simulink model "sst_cllc_dcx"  (R2026b)
settings: Solver=ode23tb  StopTime=param.sim.simlength  FixedStep=tc  MaxStep=param.glb_time.tc
values from neighbouring files (symbols this model uses):
  param = struct()    [init_model.m]
undefined symbols (not defined in the file or in its folder): cllc_dcx_param_example
libraries: fl_lib x144, nesl_utility x71, mos_simple_2th_lib x8, discrete_time_low_pass_filter x2, lithium_ion_battery x1, cllc_dcx x1, single_phase_transformer x1, dab_single_phase_pwm_modulator x1, ee_lib x1
(part 3 of 4)

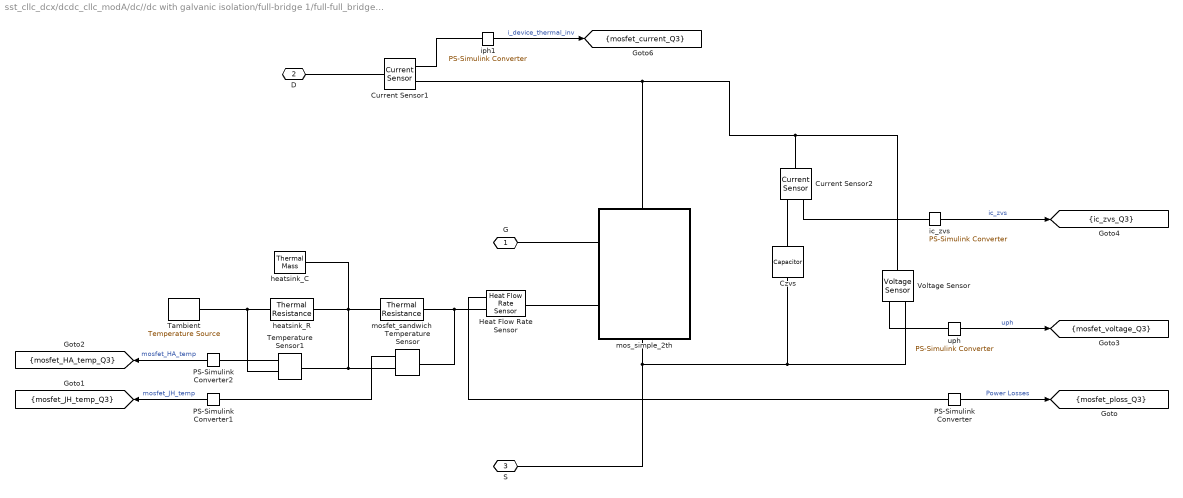
== system sst_cllc_dcx/dcdc_cllc_modA/dc//dc with galvanic isolation/full-bridge 1/full-full_bridge_ssc_mosfet_based/full_bridge_ssc_mosfet_based/mosfet_thermal_3 ==
  Current Sensor1 : fl_lib/Electrical/Electrical Sensors/Current Sensor
  Current Sensor2 : fl_lib/Electrical/Electrical Sensors/Current Sensor
  Czvs : fl_lib/Electrical/Electrical Elements/Capacitor  c=Csnubber_m F  r=Rsnubber_m Ohm  g=0 1/Ohm  i_specify=off  i_priority=None  i=0 A  i_nominal_specify=off  i_nominal_value=1  i_nominal_unit=A  v_specify=off  v_priority=None  v=0 V  v_nominal_specify=off  v_nominal_value=1  v_nominal_unit=V  vc_specify=off  vc_priority=High  vc=0 V  vc_nominal_specify=off  vc_nominal_value=1  vc_nominal_unit=V
  Heat Flow Rate Sensor : fl_lib/Thermal/Thermal Sensors/Heat Flow Rate Sensor
  PS-Simulink Converter : nesl_utility/PS-Simulink Converter  PhysicalDomain=network_engine_domain  SubClassName=ps_output  LeftPortType=input  RightPortType=output  PseudoPeriodic=off  Frequencies=[]  VectorFormat=1-D array  Unit=W  AffineConversion=off
  PS-Simulink Converter1 : nesl_utility/PS-Simulink Converter  PhysicalDomain=network_engine_domain  SubClassName=ps_output  LeftPortType=input  RightPortType=output  PseudoPeriodic=off  Frequencies=[]  VectorFormat=1-D array  Unit=degC  AffineConversion=off
  PS-Simulink Converter2 : nesl_utility/PS-Simulink Converter  PhysicalDomain=network_engine_domain  SubClassName=ps_output  LeftPortType=input  RightPortType=output  PseudoPeriodic=off  Frequencies=[]  VectorFormat=1-D array  Unit=degC  AffineConversion=off
  Tambient : fl_lib/Thermal/Thermal Sources/Temperature Source  temperature=Tambient_m degC
  Temperature Sensor : fl_lib/Thermal/Thermal Sensors/Temperature Sensor  temperature_measure=foundation.enum.MeasurementReference.difference
  Temperature Sensor1 : fl_lib/Thermal/Thermal Sensors/Temperature Sensor  temperature_measure=foundation.enum.MeasurementReference.difference
  Voltage Sensor : fl_lib/Electrical/Electrical Sensors/Voltage Sensor
  heatsink_C : fl_lib/Thermal/Thermal Elements/Thermal Mass  mass_type=foundation.enum.constant_variable.constant  mass=mass_heatsink_m kg  sp_heat=specific_heat_m J/(K*kg)  mass_min=1e-6 kg  num_ports=foundation.enum.numPorts2.one  m_specify=off  m_priority=High  m=1 kg  m_nominal_specify=off  m_nominal_value=1  m_nominal_unit=kg  T_specify=on  T_priority=High  T=DThs_init_m+Tambient_m degC  T_nominal_specify=off  T_nominal_value=1  T_nominal_unit=K  Q_specify=off  Q_priority=High  Q=0 W  Q_nominal_specify=off  Q_nominal_value=1  Q_nominal_unit=W
  heatsink_R : fl_lib/Thermal/Thermal Elements/Thermal Resistance  resistance=rth_mosfet_HA_m K/W  T_specify=off  T_priority=High  T=0 deltadegC  T_nominal_specify=off  T_nominal_value=1  T_nominal_unit=K  Q_specify=off  Q_priority=None  Q=0 W  Q_nominal_specify=off  Q_nominal_value=1  Q_nominal_unit=W
  ic_zvs : nesl_utility/PS-Simulink Converter  PhysicalDomain=network_engine_domain  SubClassName=ps_output  LeftPortType=input  RightPortType=output  PseudoPeriodic=off  Frequencies=[]  VectorFormat=1-D array  Unit=A  AffineConversion=off
  iph1 : nesl_utility/PS-Simulink Converter  PhysicalDomain=network_engine_domain  SubClassName=ps_output  LeftPortType=input  RightPortType=output  PseudoPeriodic=off  Frequencies=[]  VectorFormat=1-D array  Unit=A  AffineConversion=off
  mos_simple_2th : Subsystem
      settings: PortSchema="{\"entries\":[{\"content\":{\"sides\":[{\"content\":{\"connectorIds\":[\"LConn1\",\"LConn2\"]},\"type\":\"ConnectorPlacement.EquallySpacedRectSide\",\"uuid\":\"0c7df1d1-e739-4cca-908e-e4e85a8d5110\"},{\"content\":{\"side\":\"RIGHT\"},\"type\":\"ConnectorPlacement.EquallySpacedRectSide\",\"uuid\":\"6e0178b8-4891-4b94-aab6-d38b52a6c94b\"},{\"content\":{\"connectorIds\":[\"LConn3\"],\"side\":\"TOP\"},\"type\":\"ConnectorPlacement.EquallySpacedRectSide\",\"uuid\":\"66a82ce3-a212-45ef-89fa-79c9554ad3a2\"},{\"content\":{\"connectorIds\":[\"RConn1\"],\"side\":\"BOTTOM\"},\"type\":\"ConnectorPlacement.EquallySpacedRectSide\",\"uuid\":\"30e3dab1-9356-4de4-b881-b8bc9cf47aa5\"}]},\"type\":\"ConnectorPlacement.EquallySpacedConnector\",\"uuid\":\"69805b64-ad78-46b1-90c4-7e7bc5808829\"}],\"packageUris\":[\"http://schema.mathworks.com/mf0/Connector/R2020b\"],\"version\":\"1.0\"}"
  mosfet_sandwich : fl_lib/Thermal/Thermal Elements/Thermal Resistance  resistance=rth_mosfet_JH_m K/W  T_specify=off  T_priority=High  T=0 degC  T_nominal_specify=off  T_nominal_value=1  T_nominal_unit=K  Q_specify=off  Q_priority=None  Q=0 W  Q_nominal_specify=off  Q_nominal_value=1  Q_nominal_unit=W
  uph : nesl_utility/PS-Simulink Converter  PhysicalDomain=network_engine_domain  SubClassName=ps_output  LeftPortType=input  RightPortType=output  PseudoPeriodic=off  Frequencies=[]  VectorFormat=1-D array  Unit=V  AffineConversion=off
  G : PMIOPort  Side=Left
  D : PMIOPort  Port=2  Side=Left
  S : PMIOPort  Port=3  Side=Right
  tag scope: ic_zvs_Q3=scoped, mosfet_HA_temp_Q3=scoped, mosfet_JH_temp_Q3=scoped, mosfet_current_Q3=scoped, mosfet_ploss_Q3=scoped, mosfet_voltage_Q3=scoped
  wires:
  ic_zvs/1 -> [ic_zvs_Q3]  "ic_zvs"
  uph/1 -> [mosfet_voltage_Q3]  "uph"
  iph1/1 -> [mosfet_current_Q3]  "i_device_thermal_inv"
  PS-Simulink Converter1/1 -> [mosfet_JH_temp_Q3]  "mosfet_JH_temp"
  PS-Simulink Converter2/1 -> [mosfet_HA_temp_Q3]  "mosfet_HA_temp"
  PS-Simulink Converter/1 -> [mosfet_ploss_Q3]  "Power Losses"
  connections:
  Current Sensor2/RConn1 -- ic_zvs/LConn1
  Czvs/LConn1 -- Current Sensor2/RConn2
  Voltage Sensor/RConn1 -- uph/LConn1
  Current Sensor1/RConn1 -- iph1/LConn1
  Voltage Sensor/LConn1 -- Current Sensor1/RConn2 -- mos_simple_2th/LConn3 -- Current Sensor2/LConn1
  Current Sensor1/LConn1 -- D/RConn1
  mos_simple_2th/LConn2 -- Heat Flow Rate Sensor/LConn1
  Temperature Sensor1/RConn2 -- PS-Simulink Converter2/LConn1
  heatsink_R/RConn1 -- Tambient/LConn1 -- Temperature Sensor1/RConn1
  Temperature Sensor/RConn2 -- PS-Simulink Converter1/LConn1
  mosfet_sandwich/RConn1 -- heatsink_C/LConn1 -- heatsink_R/LConn1 -- Temperature Sensor/RConn1 -- Temperature Sensor1/LConn1
  Heat Flow Rate Sensor/RConn2 -- mosfet_sandwich/LConn1 -- Temperature Sensor/LConn1
  PS-Simulink Converter/LConn1 -- Heat Flow Rate Sensor/RConn1
  mos_simple_2th/LConn1 -- G/RConn1
  Voltage Sensor/RConn2 -- Czvs/RConn1 -- S/RConn1 -- mos_simple_2th/RConn1

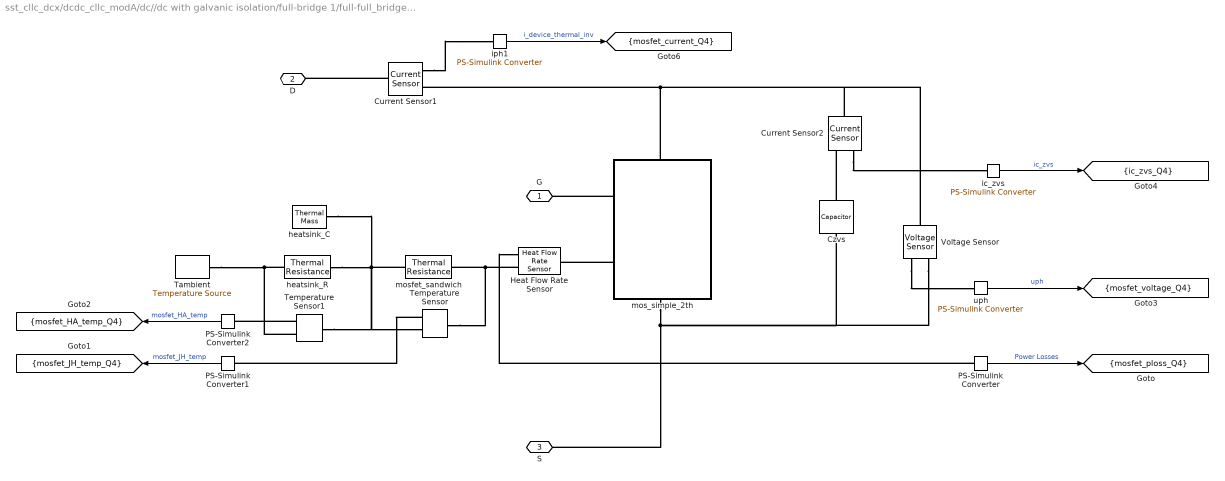
== system sst_cllc_dcx/dcdc_cllc_modA/dc//dc with galvanic isolation/full-bridge 1/full-full_bridge_ssc_mosfet_based/full_bridge_ssc_mosfet_based/mosfet_thermal_4 ==
  Current Sensor1 : fl_lib/Electrical/Electrical Sensors/Current Sensor
  Current Sensor2 : fl_lib/Electrical/Electrical Sensors/Current Sensor
  Czvs : fl_lib/Electrical/Electrical Elements/Capacitor  c=Csnubber_m F  r=Rsnubber_m Ohm  g=0 1/Ohm  i_specify=off  i_priority=None  i=0 A  i_nominal_specify=off  i_nominal_value=1  i_nominal_unit=A  v_specify=off  v_priority=None  v=0 V  v_nominal_specify=off  v_nominal_value=1  v_nominal_unit=V  vc_specify=off  vc_priority=High  vc=0 V  vc_nominal_specify=off  vc_nominal_value=1  vc_nominal_unit=V
  Heat Flow Rate Sensor : fl_lib/Thermal/Thermal Sensors/Heat Flow Rate Sensor
  PS-Simulink Converter : nesl_utility/PS-Simulink Converter  PhysicalDomain=network_engine_domain  SubClassName=ps_output  LeftPortType=input  RightPortType=output  PseudoPeriodic=off  Frequencies=[]  VectorFormat=1-D array  Unit=W  AffineConversion=off
  PS-Simulink Converter1 : nesl_utility/PS-Simulink Converter  PhysicalDomain=network_engine_domain  SubClassName=ps_output  LeftPortType=input  RightPortType=output  PseudoPeriodic=off  Frequencies=[]  VectorFormat=1-D array  Unit=degC  AffineConversion=off
  PS-Simulink Converter2 : nesl_utility/PS-Simulink Converter  PhysicalDomain=network_engine_domain  SubClassName=ps_output  LeftPortType=input  RightPortType=output  PseudoPeriodic=off  Frequencies=[]  VectorFormat=1-D array  Unit=degC  AffineConversion=off
  Tambient : fl_lib/Thermal/Thermal Sources/Temperature Source  temperature=Tambient_m degC
  Temperature Sensor : fl_lib/Thermal/Thermal Sensors/Temperature Sensor  temperature_measure=foundation.enum.MeasurementReference.difference
  Temperature Sensor1 : fl_lib/Thermal/Thermal Sensors/Temperature Sensor  temperature_measure=foundation.enum.MeasurementReference.difference
  Voltage Sensor : fl_lib/Electrical/Electrical Sensors/Voltage Sensor
  heatsink_C : fl_lib/Thermal/Thermal Elements/Thermal Mass  mass_type=foundation.enum.constant_variable.constant  mass=mass_heatsink_m kg  sp_heat=specific_heat_m J/(K*kg)  mass_min=1e-6 kg  num_ports=foundation.enum.numPorts2.one  m_specify=off  m_priority=High  m=1 kg  m_nominal_specify=off  m_nominal_value=1  m_nominal_unit=kg  T_specify=on  T_priority=High  T=DThs_init_m+Tambient_m degC  T_nominal_specify=off  T_nominal_value=1  T_nominal_unit=K  Q_specify=off  Q_priority=High  Q=0 W  Q_nominal_specify=off  Q_nominal_value=1  Q_nominal_unit=W
  heatsink_R : fl_lib/Thermal/Thermal Elements/Thermal Resistance  resistance=rth_mosfet_HA_m K/W  T_specify=off  T_priority=High  T=0 deltadegC  T_nominal_specify=off  T_nominal_value=1  T_nominal_unit=K  Q_specify=off  Q_priority=None  Q=0 W  Q_nominal_specify=off  Q_nominal_value=1  Q_nominal_unit=W
  ic_zvs : nesl_utility/PS-Simulink Converter  PhysicalDomain=network_engine_domain  SubClassName=ps_output  LeftPortType=input  RightPortType=output  PseudoPeriodic=off  Frequencies=[]  VectorFormat=1-D array  Unit=A  AffineConversion=off
  iph1 : nesl_utility/PS-Simulink Converter  PhysicalDomain=network_engine_domain  SubClassName=ps_output  LeftPortType=input  RightPortType=output  PseudoPeriodic=off  Frequencies=[]  VectorFormat=1-D array  Unit=A  AffineConversion=off
  mos_simple_2th : Subsystem
      settings: PortSchema="{\"entries\":[{\"content\":{\"sides\":[{\"content\":{\"connectorIds\":[\"LConn1\",\"LConn2\"]},\"type\":\"ConnectorPlacement.EquallySpacedRectSide\",\"uuid\":\"0c7df1d1-e739-4cca-908e-e4e85a8d5110\"},{\"content\":{\"side\":\"RIGHT\"},\"type\":\"ConnectorPlacement.EquallySpacedRectSide\",\"uuid\":\"6e0178b8-4891-4b94-aab6-d38b52a6c94b\"},{\"content\":{\"connectorIds\":[\"LConn3\"],\"side\":\"TOP\"},\"type\":\"ConnectorPlacement.EquallySpacedRectSide\",\"uuid\":\"66a82ce3-a212-45ef-89fa-79c9554ad3a2\"},{\"content\":{\"connectorIds\":[\"RConn1\"],\"side\":\"BOTTOM\"},\"type\":\"ConnectorPlacement.EquallySpacedRectSide\",\"uuid\":\"30e3dab1-9356-4de4-b881-b8bc9cf47aa5\"}]},\"type\":\"ConnectorPlacement.EquallySpacedConnector\",\"uuid\":\"69805b64-ad78-46b1-90c4-7e7bc5808829\"}],\"packageUris\":[\"http://schema.mathworks.com/mf0/Connector/R2020b\"],\"version\":\"1.0\"}"
  mosfet_sandwich : fl_lib/Thermal/Thermal Elements/Thermal Resistance  resistance=rth_mosfet_JH_m K/W  T_specify=off  T_priority=High  T=0 degC  T_nominal_specify=off  T_nominal_value=1  T_nominal_unit=K  Q_specify=off  Q_priority=None  Q=0 W  Q_nominal_specify=off  Q_nominal_value=1  Q_nominal_unit=W
  uph : nesl_utility/PS-Simulink Converter  PhysicalDomain=network_engine_domain  SubClassName=ps_output  LeftPortType=input  RightPortType=output  PseudoPeriodic=off  Frequencies=[]  VectorFormat=1-D array  Unit=V  AffineConversion=off
  G : PMIOPort  Side=Left
  D : PMIOPort  Port=2  Side=Left
  S : PMIOPort  Port=3  Side=Right
  tag scope: ic_zvs_Q4=scoped, mosfet_HA_temp_Q4=scoped, mosfet_JH_temp_Q4=scoped, mosfet_current_Q4=scoped, mosfet_ploss_Q4=scoped, mosfet_voltage_Q4=scoped
  wires:
  ic_zvs/1 -> [ic_zvs_Q4]  "ic_zvs"
  PS-Simulink Converter/1 -> [mosfet_ploss_Q4]  "Power Losses"
  PS-Simulink Converter2/1 -> [mosfet_HA_temp_Q4]  "mosfet_HA_temp"
  PS-Simulink Converter1/1 -> [mosfet_JH_temp_Q4]  "mosfet_JH_temp"
  iph1/1 -> [mosfet_current_Q4]  "i_device_thermal_inv"
  uph/1 -> [mosfet_voltage_Q4]  "uph"
  connections:
  Current Sensor2/RConn1 -- ic_zvs/LConn1
  Czvs/LConn1 -- Current Sensor2/RConn2
  Czvs/RConn1 -- Voltage Sensor/RConn2 -- mos_simple_2th/RConn1 -- S/RConn1
  mos_simple_2th/LConn1 -- G/RConn1
  PS-Simulink Converter/LConn1 -- Heat Flow Rate Sensor/RConn1
  Temperature Sensor/LConn1 -- mosfet_sandwich/LConn1 -- Heat Flow Rate Sensor/RConn2
  mosfet_sandwich/RConn1 -- heatsink_C/LConn1 -- heatsink_R/LConn1 -- Temperature Sensor1/LConn1 -- Temperature Sensor/RConn1
  Temperature Sensor/RConn2 -- PS-Simulink Converter1/LConn1
  heatsink_R/RConn1 -- Tambient/LConn1 -- Temperature Sensor1/RConn1
  Temperature Sensor1/RConn2 -- PS-Simulink Converter2/LConn1
  mos_simple_2th/LConn2 -- Heat Flow Rate Sensor/LConn1
  Current Sensor1/LConn1 -- D/RConn1
  Current Sensor2/LConn1 -- Voltage Sensor/LConn1 -- mos_simple_2th/LConn3 -- Current Sensor1/RConn2
  Current Sensor1/RConn1 -- iph1/LConn1
  Voltage Sensor/RConn1 -- uph/LConn1

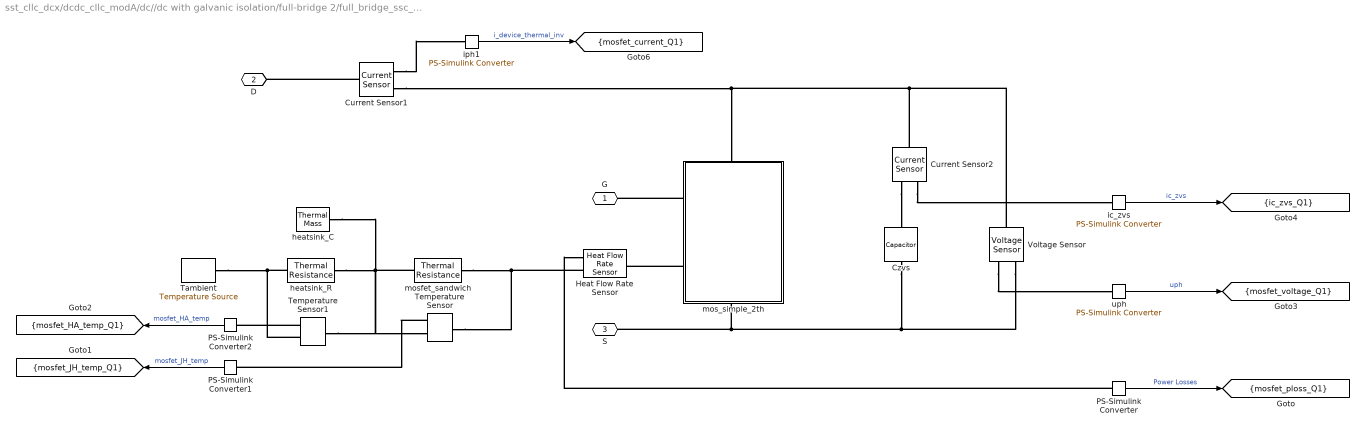
== system sst_cllc_dcx/dcdc_cllc_modA/dc//dc with galvanic isolation/full-bridge 2/full_bridge_ssc_mosfet_based/full_bridge_ssc_mosfet_based/mosfet_thermal_1 ==
  Current Sensor1 : fl_lib/Electrical/Electrical Sensors/Current Sensor
  Current Sensor2 : fl_lib/Electrical/Electrical Sensors/Current Sensor
  Czvs : fl_lib/Electrical/Electrical Elements/Capacitor  c=Csnubber_m F  r=Rsnubber_m Ohm  g=0 1/Ohm  i_specify=off  i_priority=None  i=0 A  i_nominal_specify=off  i_nominal_value=1  i_nominal_unit=A  v_specify=off  v_priority=None  v=0 V  v_nominal_specify=off  v_nominal_value=1  v_nominal_unit=V  vc_specify=off  vc_priority=High  vc=0 V  vc_nominal_specify=off  vc_nominal_value=1  vc_nominal_unit=V
  Heat Flow Rate Sensor : fl_lib/Thermal/Thermal Sensors/Heat Flow Rate Sensor
  PS-Simulink Converter : nesl_utility/PS-Simulink Converter  PhysicalDomain=network_engine_domain  SubClassName=ps_output  LeftPortType=input  RightPortType=output  PseudoPeriodic=off  Frequencies=[]  VectorFormat=1-D array  Unit=W  AffineConversion=off
  PS-Simulink Converter1 : nesl_utility/PS-Simulink Converter  PhysicalDomain=network_engine_domain  SubClassName=ps_output  LeftPortType=input  RightPortType=output  PseudoPeriodic=off  Frequencies=[]  VectorFormat=1-D array  Unit=degC  AffineConversion=off
  PS-Simulink Converter2 : nesl_utility/PS-Simulink Converter  PhysicalDomain=network_engine_domain  SubClassName=ps_output  LeftPortType=input  RightPortType=output  PseudoPeriodic=off  Frequencies=[]  VectorFormat=1-D array  Unit=degC  AffineConversion=off
  Tambient : fl_lib/Thermal/Thermal Sources/Temperature Source  temperature=Tambient_m degC
  Temperature Sensor : fl_lib/Thermal/Thermal Sensors/Temperature Sensor  temperature_measure=foundation.enum.MeasurementReference.difference
  Temperature Sensor1 : fl_lib/Thermal/Thermal Sensors/Temperature Sensor  temperature_measure=foundation.enum.MeasurementReference.difference
  Voltage Sensor : fl_lib/Electrical/Electrical Sensors/Voltage Sensor
  heatsink_C : fl_lib/Thermal/Thermal Elements/Thermal Mass  mass_type=foundation.enum.constant_variable.constant  mass=mass_heatsink_m kg  sp_heat=specific_heat_m J/(K*kg)  mass_min=1e-6 kg  num_ports=foundation.enum.numPorts2.one  m_specify=off  m_priority=High  m=1 kg  m_nominal_specify=off  m_nominal_value=1  m_nominal_unit=kg  T_specify=on  T_priority=High  T=DThs_init_m+Tambient_m degC  T_nominal_specify=off  T_nominal_value=1  T_nominal_unit=K  Q_specify=off  Q_priority=High  Q=0 W  Q_nominal_specify=off  Q_nominal_value=1  Q_nominal_unit=W
  heatsink_R : fl_lib/Thermal/Thermal Elements/Thermal Resistance  resistance=rth_mosfet_HA_m K/W  T_specify=off  T_priority=High  T=0 deltadegC  T_nominal_specify=off  T_nominal_value=1  T_nominal_unit=K  Q_specify=off  Q_priority=None  Q=0 W  Q_nominal_specify=off  Q_nominal_value=1  Q_nominal_unit=W
  ic_zvs : nesl_utility/PS-Simulink Converter  PhysicalDomain=network_engine_domain  SubClassName=ps_output  LeftPortType=input  RightPortType=output  PseudoPeriodic=off  Frequencies=[]  VectorFormat=1-D array  Unit=A  AffineConversion=off
  iph1 : nesl_utility/PS-Simulink Converter  PhysicalDomain=network_engine_domain  SubClassName=ps_output  LeftPortType=input  RightPortType=output  PseudoPeriodic=off  Frequencies=[]  VectorFormat=1-D array  Unit=A  AffineConversion=off
  mos_simple_2th : Subsystem
      settings: PortSchema="{\"entries\":[{\"content\":{\"sides\":[{\"content\":{\"connectorIds\":[\"LConn1\",\"LConn2\"]},\"type\":\"ConnectorPlacement.EquallySpacedRectSide\",\"uuid\":\"0c7df1d1-e739-4cca-908e-e4e85a8d5110\"},{\"content\":{\"side\":\"RIGHT\"},\"type\":\"ConnectorPlacement.EquallySpacedRectSide\",\"uuid\":\"6e0178b8-4891-4b94-aab6-d38b52a6c94b\"},{\"content\":{\"connectorIds\":[\"LConn3\"],\"side\":\"TOP\"},\"type\":\"ConnectorPlacement.EquallySpacedRectSide\",\"uuid\":\"66a82ce3-a212-45ef-89fa-79c9554ad3a2\"},{\"content\":{\"connectorIds\":[\"RConn1\"],\"side\":\"BOTTOM\"},\"type\":\"ConnectorPlacement.EquallySpacedRectSide\",\"uuid\":\"30e3dab1-9356-4de4-b881-b8bc9cf47aa5\"}]},\"type\":\"ConnectorPlacement.EquallySpacedConnector\",\"uuid\":\"69805b64-ad78-46b1-90c4-7e7bc5808829\"}],\"packageUris\":[\"http://schema.mathworks.com/mf0/Connector/R2020b\"],\"version\":\"1.0\"}"
  mosfet_sandwich : fl_lib/Thermal/Thermal Elements/Thermal Resistance  resistance=rth_mosfet_JH_m K/W  T_specify=off  T_priority=High  T=0 degC  T_nominal_specify=off  T_nominal_value=1  T_nominal_unit=K  Q_specify=off  Q_priority=None  Q=0 W  Q_nominal_specify=off  Q_nominal_value=1  Q_nominal_unit=W
  uph : nesl_utility/PS-Simulink Converter  PhysicalDomain=network_engine_domain  SubClassName=ps_output  LeftPortType=input  RightPortType=output  PseudoPeriodic=off  Frequencies=[]  VectorFormat=1-D array  Unit=V  AffineConversion=off
  G : PMIOPort  Side=Left
  D : PMIOPort  Port=2  Side=Left
  S : PMIOPort  Port=3  Side=Right
  tag scope: ic_zvs_Q1=scoped, mosfet_HA_temp_Q1=scoped, mosfet_JH_temp_Q1=scoped, mosfet_current_Q1=scoped, mosfet_ploss_Q1=scoped, mosfet_voltage_Q1=scoped
  wires:
  ic_zvs/1 -> [ic_zvs_Q1]  "ic_zvs"
  uph/1 -> [mosfet_voltage_Q1]  "uph"
  iph1/1 -> [mosfet_current_Q1]  "i_device_thermal_inv"
  PS-Simulink Converter1/1 -> [mosfet_JH_temp_Q1]  "mosfet_JH_temp"
  PS-Simulink Converter2/1 -> [mosfet_HA_temp_Q1]  "mosfet_HA_temp"
  PS-Simulink Converter/1 -> [mosfet_ploss_Q1]  "Power Losses"
  connections:
  Current Sensor2/RConn1 -- ic_zvs/LConn1
  Current Sensor2/RConn2 -- Czvs/LConn1
  Voltage Sensor/RConn1 -- uph/LConn1
  Current Sensor1/RConn1 -- iph1/LConn1
  Voltage Sensor/LConn1 -- Current Sensor2/LConn1 -- Current Sensor1/RConn2 -- mos_simple_2th/LConn3
  Current Sensor1/LConn1 -- D/RConn1
  mos_simple_2th/LConn2 -- Heat Flow Rate Sensor/LConn1
  Temperature Sensor1/RConn2 -- PS-Simulink Converter2/LConn1
  Temperature Sensor1/RConn1 -- heatsink_R/RConn1 -- Tambient/LConn1
  Temperature Sensor/RConn2 -- PS-Simulink Converter1/LConn1
  heatsink_C/LConn1 -- heatsink_R/LConn1 -- mosfet_sandwich/RConn1 -- Temperature Sensor/RConn1 -- Temperature Sensor1/LConn1
  Heat Flow Rate Sensor/RConn2 -- mosfet_sandwich/LConn1 -- Temperature Sensor/LConn1
  PS-Simulink Converter/LConn1 -- Heat Flow Rate Sensor/RConn1
  mos_simple_2th/LConn1 -- G/RConn1
  Voltage Sensor/RConn2 -- S/RConn1 -- mos_simple_2th/RConn1 -- Czvs/RConn1

== system sst_cllc_dcx/dcdc_cllc_modA/dc//dc with galvanic isolation/full-bridge 2/full_bridge_ssc_mosfet_based/full_bridge_ssc_mosfet_based/mosfet_thermal_2 ==
  Current Sensor1 : fl_lib/Electrical/Electrical Sensors/Current Sensor
  Current Sensor2 : fl_lib/Electrical/Electrical Sensors/Current Sensor
  Czvs : fl_lib/Electrical/Electrical Elements/Capacitor  c=Csnubber_m F  r=Rsnubber_m Ohm  g=0 1/Ohm  i_specify=off  i_priority=None  i=0 A  i_nominal_specify=off  i_nominal_value=1  i_nominal_unit=A  v_specify=off  v_priority=None  v=0 V  v_nominal_specify=off  v_nominal_value=1  v_nominal_unit=V  vc_specify=off  vc_priority=High  vc=0 V  vc_nominal_specify=off  vc_nominal_value=1  vc_nominal_unit=V
  Heat Flow Rate Sensor : fl_lib/Thermal/Thermal Sensors/Heat Flow Rate Sensor
  PS-Simulink Converter : nesl_utility/PS-Simulink Converter  PhysicalDomain=network_engine_domain  SubClassName=ps_output  LeftPortType=input  RightPortType=output  PseudoPeriodic=off  Frequencies=[]  VectorFormat=1-D array  Unit=W  AffineConversion=off
  PS-Simulink Converter1 : nesl_utility/PS-Simulink Converter  PhysicalDomain=network_engine_domain  SubClassName=ps_output  LeftPortType=input  RightPortType=output  PseudoPeriodic=off  Frequencies=[]  VectorFormat=1-D array  Unit=degC  AffineConversion=off
  PS-Simulink Converter2 : nesl_utility/PS-Simulink Converter  PhysicalDomain=network_engine_domain  SubClassName=ps_output  LeftPortType=input  RightPortType=output  PseudoPeriodic=off  Frequencies=[]  VectorFormat=1-D array  Unit=degC  AffineConversion=off
  Tambient : fl_lib/Thermal/Thermal Sources/Temperature Source  temperature=Tambient_m degC
  Temperature Sensor : fl_lib/Thermal/Thermal Sensors/Temperature Sensor  temperature_measure=foundation.enum.MeasurementReference.difference
  Temperature Sensor1 : fl_lib/Thermal/Thermal Sensors/Temperature Sensor  temperature_measure=foundation.enum.MeasurementReference.difference
  Voltage Sensor : fl_lib/Electrical/Electrical Sensors/Voltage Sensor
  heatsink_C : fl_lib/Thermal/Thermal Elements/Thermal Mass  mass_type=foundation.enum.constant_variable.constant  mass=mass_heatsink_m kg  sp_heat=specific_heat_m J/(K*kg)  mass_min=1e-6 kg  num_ports=foundation.enum.numPorts2.one  m_specify=off  m_priority=High  m=1 kg  m_nominal_specify=off  m_nominal_value=1  m_nominal_unit=kg  T_specify=on  T_priority=High  T=DThs_init_m+Tambient_m degC  T_nominal_specify=off  T_nominal_value=1  T_nominal_unit=K  Q_specify=off  Q_priority=High  Q=0 W  Q_nominal_specify=off  Q_nominal_value=1  Q_nominal_unit=W
  heatsink_R : fl_lib/Thermal/Thermal Elements/Thermal Resistance  resistance=rth_mosfet_HA_m K/W  T_specify=off  T_priority=High  T=0 deltadegC  T_nominal_specify=off  T_nominal_value=1  T_nominal_unit=K  Q_specify=off  Q_priority=None  Q=0 W  Q_nominal_specify=off  Q_nominal_value=1  Q_nominal_unit=W
  ic_zvs : nesl_utility/PS-Simulink Converter  PhysicalDomain=network_engine_domain  SubClassName=ps_output  LeftPortType=input  RightPortType=output  PseudoPeriodic=off  Frequencies=[]  VectorFormat=1-D array  Unit=A  AffineConversion=off
  iph1 : nesl_utility/PS-Simulink Converter  PhysicalDomain=network_engine_domain  SubClassName=ps_output  LeftPortType=input  RightPortType=output  PseudoPeriodic=off  Frequencies=[]  VectorFormat=1-D array  Unit=A  AffineConversion=off
  mos_simple_2th : Subsystem
      settings: PortSchema="{\"entries\":[{\"content\":{\"sides\":[{\"content\":{\"connectorIds\":[\"LConn1\",\"LConn2\"]},\"type\":\"ConnectorPlacement.EquallySpacedRectSide\",\"uuid\":\"0c7df1d1-e739-4cca-908e-e4e85a8d5110\"},{\"content\":{\"side\":\"RIGHT\"},\"type\":\"ConnectorPlacement.EquallySpacedRectSide\",\"uuid\":\"6e0178b8-4891-4b94-aab6-d38b52a6c94b\"},{\"content\":{\"connectorIds\":[\"LConn3\"],\"side\":\"TOP\"},\"type\":\"ConnectorPlacement.EquallySpacedRectSide\",\"uuid\":\"66a82ce3-a212-45ef-89fa-79c9554ad3a2\"},{\"content\":{\"connectorIds\":[\"RConn1\"],\"side\":\"BOTTOM\"},\"type\":\"ConnectorPlacement.EquallySpacedRectSide\",\"uuid\":\"30e3dab1-9356-4de4-b881-b8bc9cf47aa5\"}]},\"type\":\"ConnectorPlacement.EquallySpacedConnector\",\"uuid\":\"69805b64-ad78-46b1-90c4-7e7bc5808829\"}],\"packageUris\":[\"http://schema.mathworks.com/mf0/Connector/R2020b\"],\"version\":\"1.0\"}"
  mosfet_sandwich : fl_lib/Thermal/Thermal Elements/Thermal Resistance  resistance=rth_mosfet_JH_m K/W  T_specify=off  T_priority=High  T=0 degC  T_nominal_specify=off  T_nominal_value=1  T_nominal_unit=K  Q_specify=off  Q_priority=None  Q=0 W  Q_nominal_specify=off  Q_nominal_value=1  Q_nominal_unit=W
  uph : nesl_utility/PS-Simulink Converter  PhysicalDomain=network_engine_domain  SubClassName=ps_output  LeftPortType=input  RightPortType=output  PseudoPeriodic=off  Frequencies=[]  VectorFormat=1-D array  Unit=V  AffineConversion=off
  G : PMIOPort  Side=Left
  D : PMIOPort  Port=2  Side=Left
  S : PMIOPort  Port=3  Side=Right
  tag scope: ic_zvs_Q2=scoped, mosfet_HA_temp_Q2=scoped, mosfet_JH_temp_Q2=scoped, mosfet_current_Q2=scoped, mosfet_ploss_Q2=scoped, mosfet_voltage_Q2=scoped
  wires:
  ic_zvs/1 -> [ic_zvs_Q2]  "ic_zvs"
  PS-Simulink Converter/1 -> [mosfet_ploss_Q2]  "Power Losses"
  PS-Simulink Converter2/1 -> [mosfet_HA_temp_Q2]  "mosfet_HA_temp"
  PS-Simulink Converter1/1 -> [mosfet_JH_temp_Q2]  "mosfet_JH_temp"
  iph1/1 -> [mosfet_current_Q2]  "i_device_thermal_inv"
  uph/1 -> [mosfet_voltage_Q2]  "uph"
  connections:
  Current Sensor2/RConn1 -- ic_zvs/LConn1
  Czvs/LConn1 -- Current Sensor2/RConn2
  Czvs/RConn1 -- mos_simple_2th/RConn1 -- S/RConn1 -- Voltage Sensor/RConn2
  mos_simple_2th/LConn1 -- G/RConn1
  PS-Simulink Converter/LConn1 -- Heat Flow Rate Sensor/RConn1
  Temperature Sensor/LConn1 -- mosfet_sandwich/LConn1 -- Heat Flow Rate Sensor/RConn2
  heatsink_R/LConn1 -- heatsink_C/LConn1 -- mosfet_sandwich/RConn1 -- Temperature Sensor/RConn1 -- Temperature Sensor1/LConn1
  Temperature Sensor/RConn2 -- PS-Simulink Converter1/LConn1
  Tambient/LConn1 -- heatsink_R/RConn1 -- Temperature Sensor1/RConn1
  Temperature Sensor1/RConn2 -- PS-Simulink Converter2/LConn1
  mos_simple_2th/LConn2 -- Heat Flow Rate Sensor/LConn1
  Current Sensor1/LConn1 -- D/RConn1
  Current Sensor2/LConn1 -- Voltage Sensor/LConn1 -- mos_simple_2th/LConn3 -- Current Sensor1/RConn2
  Current Sensor1/RConn1 -- iph1/LConn1
  Voltage Sensor/RConn1 -- uph/LConn1

== system sst_cllc_dcx/dcdc_cllc_modA/dc//dc with galvanic isolation/full-bridge 2/full_bridge_ssc_mosfet_based/full_bridge_ssc_mosfet_based/mosfet_thermal_3 ==
  Current Sensor1 : fl_lib/Electrical/Electrical Sensors/Current Sensor
  Current Sensor2 : fl_lib/Electrical/Electrical Sensors/Current Sensor
  Czvs : fl_lib/Electrical/Electrical Elements/Capacitor  c=Csnubber_m F  r=Rsnubber_m Ohm  g=0 1/Ohm  i_specify=off  i_priority=None  i=0 A  i_nominal_specify=off  i_nominal_value=1  i_nominal_unit=A  v_specify=off  v_priority=None  v=0 V  v_nominal_specify=off  v_nominal_value=1  v_nominal_unit=V  vc_specify=off  vc_priority=High  vc=0 V  vc_nominal_specify=off  vc_nominal_value=1  vc_nominal_unit=V
  Heat Flow Rate Sensor : fl_lib/Thermal/Thermal Sensors/Heat Flow Rate Sensor
  PS-Simulink Converter : nesl_utility/PS-Simulink Converter  PhysicalDomain=network_engine_domain  SubClassName=ps_output  LeftPortType=input  RightPortType=output  PseudoPeriodic=off  Frequencies=[]  VectorFormat=1-D array  Unit=W  AffineConversion=off
  PS-Simulink Converter1 : nesl_utility/PS-Simulink Converter  PhysicalDomain=network_engine_domain  SubClassName=ps_output  LeftPortType=input  RightPortType=output  PseudoPeriodic=off  Frequencies=[]  VectorFormat=1-D array  Unit=degC  AffineConversion=off
  PS-Simulink Converter2 : nesl_utility/PS-Simulink Converter  PhysicalDomain=network_engine_domain  SubClassName=ps_output  LeftPortType=input  RightPortType=output  PseudoPeriodic=off  Frequencies=[]  VectorFormat=1-D array  Unit=degC  AffineConversion=off
  Tambient : fl_lib/Thermal/Thermal Sources/Temperature Source  temperature=Tambient_m degC
  Temperature Sensor : fl_lib/Thermal/Thermal Sensors/Temperature Sensor  temperature_measure=foundation.enum.MeasurementReference.difference
  Temperature Sensor1 : fl_lib/Thermal/Thermal Sensors/Temperature Sensor  temperature_measure=foundation.enum.MeasurementReference.difference
  Voltage Sensor : fl_lib/Electrical/Electrical Sensors/Voltage Sensor
  heatsink_C : fl_lib/Thermal/Thermal Elements/Thermal Mass  mass_type=foundation.enum.constant_variable.constant  mass=mass_heatsink_m kg  sp_heat=specific_heat_m J/(K*kg)  mass_min=1e-6 kg  num_ports=foundation.enum.numPorts2.one  m_specify=off  m_priority=High  m=1 kg  m_nominal_specify=off  m_nominal_value=1  m_nominal_unit=kg  T_specify=on  T_priority=High  T=DThs_init_m+Tambient_m degC  T_nominal_specify=off  T_nominal_value=1  T_nominal_unit=K  Q_specify=off  Q_priority=High  Q=0 W  Q_nominal_specify=off  Q_nominal_value=1  Q_nominal_unit=W
  heatsink_R : fl_lib/Thermal/Thermal Elements/Thermal Resistance  resistance=rth_mosfet_HA_m K/W  T_specify=off  T_priority=High  T=0 deltadegC  T_nominal_specify=off  T_nominal_value=1  T_nominal_unit=K  Q_specify=off  Q_priority=None  Q=0 W  Q_nominal_specify=off  Q_nominal_value=1  Q_nominal_unit=W
  ic_zvs : nesl_utility/PS-Simulink Converter  PhysicalDomain=network_engine_domain  SubClassName=ps_output  LeftPortType=input  RightPortType=output  PseudoPeriodic=off  Frequencies=[]  VectorFormat=1-D array  Unit=A  AffineConversion=off
  iph1 : nesl_utility/PS-Simulink Converter  PhysicalDomain=network_engine_domain  SubClassName=ps_output  LeftPortType=input  RightPortType=output  PseudoPeriodic=off  Frequencies=[]  VectorFormat=1-D array  Unit=A  AffineConversion=off
  mos_simple_2th : Subsystem
      settings: PortSchema="{\"entries\":[{\"content\":{\"sides\":[{\"content\":{\"connectorIds\":[\"LConn1\",\"LConn2\"]},\"type\":\"ConnectorPlacement.EquallySpacedRectSide\",\"uuid\":\"0c7df1d1-e739-4cca-908e-e4e85a8d5110\"},{\"content\":{\"side\":\"RIGHT\"},\"type\":\"ConnectorPlacement.EquallySpacedRectSide\",\"uuid\":\"6e0178b8-4891-4b94-aab6-d38b52a6c94b\"},{\"content\":{\"connectorIds\":[\"LConn3\"],\"side\":\"TOP\"},\"type\":\"ConnectorPlacement.EquallySpacedRectSide\",\"uuid\":\"66a82ce3-a212-45ef-89fa-79c9554ad3a2\"},{\"content\":{\"connectorIds\":[\"RConn1\"],\"side\":\"BOTTOM\"},\"type\":\"ConnectorPlacement.EquallySpacedRectSide\",\"uuid\":\"30e3dab1-9356-4de4-b881-b8bc9cf47aa5\"}]},\"type\":\"ConnectorPlacement.EquallySpacedConnector\",\"uuid\":\"69805b64-ad78-46b1-90c4-7e7bc5808829\"}],\"packageUris\":[\"http://schema.mathworks.com/mf0/Connector/R2020b\"],\"version\":\"1.0\"}"
  mosfet_sandwich : fl_lib/Thermal/Thermal Elements/Thermal Resistance  resistance=rth_mosfet_JH_m K/W  T_specify=off  T_priority=High  T=0 degC  T_nominal_specify=off  T_nominal_value=1  T_nominal_unit=K  Q_specify=off  Q_priority=None  Q=0 W  Q_nominal_specify=off  Q_nominal_value=1  Q_nominal_unit=W
  uph : nesl_utility/PS-Simulink Converter  PhysicalDomain=network_engine_domain  SubClassName=ps_output  LeftPortType=input  RightPortType=output  PseudoPeriodic=off  Frequencies=[]  VectorFormat=1-D array  Unit=V  AffineConversion=off
  G : PMIOPort  Side=Left
  D : PMIOPort  Port=2  Side=Left
  S : PMIOPort  Port=3  Side=Right
  tag scope: ic_zvs_Q3=scoped, mosfet_HA_temp_Q3=scoped, mosfet_JH_temp_Q3=scoped, mosfet_current_Q3=scoped, mosfet_ploss_Q3=scoped, mosfet_voltage_Q3=scoped
  wires:
  ic_zvs/1 -> [ic_zvs_Q3]  "ic_zvs"
  uph/1 -> [mosfet_voltage_Q3]  "uph"
  iph1/1 -> [mosfet_current_Q3]  "i_device_thermal_inv"
  PS-Simulink Converter1/1 -> [mosfet_JH_temp_Q3]  "mosfet_JH_temp"
  PS-Simulink Converter2/1 -> [mosfet_HA_temp_Q3]  "mosfet_HA_temp"
  PS-Simulink Converter/1 -> [mosfet_ploss_Q3]  "Power Losses"
  connections:
  Current Sensor2/RConn1 -- ic_zvs/LConn1
  Czvs/LConn1 -- Current Sensor2/RConn2
  Voltage Sensor/RConn1 -- uph/LConn1
  Current Sensor1/RConn1 -- iph1/LConn1
  Voltage Sensor/LConn1 -- mos_simple_2th/LConn3 -- Current Sensor1/RConn2 -- Current Sensor2/LConn1
  Current Sensor1/LConn1 -- D/RConn1
  mos_simple_2th/LConn2 -- Heat Flow Rate Sensor/LConn1
  Temperature Sensor1/RConn2 -- PS-Simulink Converter2/LConn1
  heatsink_R/RConn1 -- Tambient/LConn1 -- Temperature Sensor1/RConn1
  Temperature Sensor/RConn2 -- PS-Simulink Converter1/LConn1
  mosfet_sandwich/RConn1 -- heatsink_C/LConn1 -- heatsink_R/LConn1 -- Temperature Sensor/RConn1 -- Temperature Sensor1/LConn1
  Heat Flow Rate Sensor/RConn2 -- mosfet_sandwich/LConn1 -- Temperature Sensor/LConn1
  PS-Simulink Converter/LConn1 -- Heat Flow Rate Sensor/RConn1
  mos_simple_2th/LConn1 -- G/RConn1
  Voltage Sensor/RConn2 -- Czvs/RConn1 -- mos_simple_2th/RConn1 -- S/RConn1

== system sst_cllc_dcx/dcdc_cllc_modA/dc//dc with galvanic isolation/full-bridge 2/full_bridge_ssc_mosfet_based/full_bridge_ssc_mosfet_based/mosfet_thermal_4 ==
  Current Sensor1 : fl_lib/Electrical/Electrical Sensors/Current Sensor
  Current Sensor2 : fl_lib/Electrical/Electrical Sensors/Current Sensor
  Czvs : fl_lib/Electrical/Electrical Elements/Capacitor  c=Csnubber_m F  r=Rsnubber_m Ohm  g=0 1/Ohm  i_specify=off  i_priority=None  i=0 A  i_nominal_specify=off  i_nominal_value=1  i_nominal_unit=A  v_specify=off  v_priority=None  v=0 V  v_nominal_specify=off  v_nominal_value=1  v_nominal_unit=V  vc_specify=off  vc_priority=High  vc=0 V  vc_nominal_specify=off  vc_nominal_value=1  vc_nominal_unit=V
  Heat Flow Rate Sensor : fl_lib/Thermal/Thermal Sensors/Heat Flow Rate Sensor
  PS-Simulink Converter : nesl_utility/PS-Simulink Converter  PhysicalDomain=network_engine_domain  SubClassName=ps_output  LeftPortType=input  RightPortType=output  PseudoPeriodic=off  Frequencies=[]  VectorFormat=1-D array  Unit=W  AffineConversion=off
  PS-Simulink Converter1 : nesl_utility/PS-Simulink Converter  PhysicalDomain=network_engine_domain  SubClassName=ps_output  LeftPortType=input  RightPortType=output  PseudoPeriodic=off  Frequencies=[]  VectorFormat=1-D array  Unit=degC  AffineConversion=off
  PS-Simulink Converter2 : nesl_utility/PS-Simulink Converter  PhysicalDomain=network_engine_domain  SubClassName=ps_output  LeftPortType=input  RightPortType=output  PseudoPeriodic=off  Frequencies=[]  VectorFormat=1-D array  Unit=degC  AffineConversion=off
  Tambient : fl_lib/Thermal/Thermal Sources/Temperature Source  temperature=Tambient_m degC
  Temperature Sensor : fl_lib/Thermal/Thermal Sensors/Temperature Sensor  temperature_measure=foundation.enum.MeasurementReference.difference
  Temperature Sensor1 : fl_lib/Thermal/Thermal Sensors/Temperature Sensor  temperature_measure=foundation.enum.MeasurementReference.difference
  Voltage Sensor : fl_lib/Electrical/Electrical Sensors/Voltage Sensor
  heatsink_C : fl_lib/Thermal/Thermal Elements/Thermal Mass  mass_type=foundation.enum.constant_variable.constant  mass=mass_heatsink_m kg  sp_heat=specific_heat_m J/(K*kg)  mass_min=1e-6 kg  num_ports=foundation.enum.numPorts2.one  m_specify=off  m_priority=High  m=1 kg  m_nominal_specify=off  m_nominal_value=1  m_nominal_unit=kg  T_specify=on  T_priority=High  T=DThs_init_m+Tambient_m degC  T_nominal_specify=off  T_nominal_value=1  T_nominal_unit=K  Q_specify=off  Q_priority=High  Q=0 W  Q_nominal_specify=off  Q_nominal_value=1  Q_nominal_unit=W
  heatsink_R : fl_lib/Thermal/Thermal Elements/Thermal Resistance  resistance=rth_mosfet_HA_m K/W  T_specify=off  T_priority=High  T=0 deltadegC  T_nominal_specify=off  T_nominal_value=1  T_nominal_unit=K  Q_specify=off  Q_priority=None  Q=0 W  Q_nominal_specify=off  Q_nominal_value=1  Q_nominal_unit=W
  ic_zvs : nesl_utility/PS-Simulink Converter  PhysicalDomain=network_engine_domain  SubClassName=ps_output  LeftPortType=input  RightPortType=output  PseudoPeriodic=off  Frequencies=[]  VectorFormat=1-D array  Unit=A  AffineConversion=off
  iph1 : nesl_utility/PS-Simulink Converter  PhysicalDomain=network_engine_domain  SubClassName=ps_output  LeftPortType=input  RightPortType=output  PseudoPeriodic=off  Frequencies=[]  VectorFormat=1-D array  Unit=A  AffineConversion=off
  mos_simple_2th : Subsystem
      settings: PortSchema="{\"entries\":[{\"content\":{\"sides\":[{\"content\":{\"connectorIds\":[\"LConn1\",\"LConn2\"]},\"type\":\"ConnectorPlacement.EquallySpacedRectSide\",\"uuid\":\"0c7df1d1-e739-4cca-908e-e4e85a8d5110\"},{\"content\":{\"side\":\"RIGHT\"},\"type\":\"ConnectorPlacement.EquallySpacedRectSide\",\"uuid\":\"6e0178b8-4891-4b94-aab6-d38b52a6c94b\"},{\"content\":{\"connectorIds\":[\"LConn3\"],\"side\":\"TOP\"},\"type\":\"ConnectorPlacement.EquallySpacedRectSide\",\"uuid\":\"66a82ce3-a212-45ef-89fa-79c9554ad3a2\"},{\"content\":{\"connectorIds\":[\"RConn1\"],\"side\":\"BOTTOM\"},\"type\":\"ConnectorPlacement.EquallySpacedRectSide\",\"uuid\":\"30e3dab1-9356-4de4-b881-b8bc9cf47aa5\"}]},\"type\":\"ConnectorPlacement.EquallySpacedConnector\",\"uuid\":\"69805b64-ad78-46b1-90c4-7e7bc5808829\"}],\"packageUris\":[\"http://schema.mathworks.com/mf0/Connector/R2020b\"],\"version\":\"1.0\"}"
  mosfet_sandwich : fl_lib/Thermal/Thermal Elements/Thermal Resistance  resistance=rth_mosfet_JH_m K/W  T_specify=off  T_priority=High  T=0 degC  T_nominal_specify=off  T_nominal_value=1  T_nominal_unit=K  Q_specify=off  Q_priority=None  Q=0 W  Q_nominal_specify=off  Q_nominal_value=1  Q_nominal_unit=W
  uph : nesl_utility/PS-Simulink Converter  PhysicalDomain=network_engine_domain  SubClassName=ps_output  LeftPortType=input  RightPortType=output  PseudoPeriodic=off  Frequencies=[]  VectorFormat=1-D array  Unit=V  AffineConversion=off
  G : PMIOPort  Side=Left
  D : PMIOPort  Port=2  Side=Left
  S : PMIOPort  Port=3  Side=Right
  tag scope: ic_zvs_Q4=scoped, mosfet_HA_temp_Q4=scoped, mosfet_JH_temp_Q4=scoped, mosfet_current_Q4=scoped, mosfet_ploss_Q4=scoped, mosfet_voltage_Q4=scoped
  wires:
  ic_zvs/1 -> [ic_zvs_Q4]  "ic_zvs"
  PS-Simulink Converter/1 -> [mosfet_ploss_Q4]  "Power Losses"
  PS-Simulink Converter2/1 -> [mosfet_HA_temp_Q4]  "mosfet_HA_temp"
  PS-Simulink Converter1/1 -> [mosfet_JH_temp_Q4]  "mosfet_JH_temp"
  iph1/1 -> [mosfet_current_Q4]  "i_device_thermal_inv"
  uph/1 -> [mosfet_voltage_Q4]  "uph"
  connections:
  Current Sensor2/RConn1 -- ic_zvs/LConn1
  Czvs/LConn1 -- Current Sensor2/RConn2
  Czvs/RConn1 -- Voltage Sensor/RConn2 -- mos_simple_2th/RConn1 -- S/RConn1
  mos_simple_2th/LConn1 -- G/RConn1
  PS-Simulink Converter/LConn1 -- Heat Flow Rate Sensor/RConn1
  Temperature Sensor/LConn1 -- mosfet_sandwich/LConn1 -- Heat Flow Rate Sensor/RConn2
  mosfet_sandwich/RConn1 -- heatsink_C/LConn1 -- heatsink_R/LConn1 -- Temperature Sensor1/LConn1 -- Temperature Sensor/RConn1
  Temperature Sensor/RConn2 -- PS-Simulink Converter1/LConn1
  heatsink_R/RConn1 -- Tambient/LConn1 -- Temperature Sensor1/RConn1
  Temperature Sensor1/RConn2 -- PS-Simulink Converter2/LConn1
  mos_simple_2th/LConn2 -- Heat Flow Rate Sensor/LConn1
  Current Sensor1/LConn1 -- D/RConn1
  Current Sensor2/LConn1 -- Voltage Sensor/LConn1 -- mos_simple_2th/LConn3 -- Current Sensor1/RConn2
  Current Sensor1/RConn1 -- iph1/LConn1
  Voltage Sensor/RConn1 -- uph/LConn1

== system sst_cllc_dcx/dcdc_cllc_modA/dc//dc with galvanic isolation/full-bridge 1/full-full_bridge_ssc_mosfet_based/full_bridge_ssc_mosfet_based/mosfet_thermal_1/mos_simple_2th ==
  PS Terminator{,1..3} (4 alike) : fl_lib/Physical Signals/Sinks/PS Terminator
  mos_simple_2th : mos_simple_2th_lib/MOS_SIMPLE_2TH Simplified power MOSFET + antiparallel diode, two thermal ports  Rds_on=Rds_on_m Ohm  alpha_R=0 1/K  Tj_ref=398.15 K  Roff=1e7 Ohm  Vf=Vdon_diode_m V  Rd=Rdon_diode_m Ohm  two_die=1  G_th=0.5  Eon_ref=Eon_m J  Eoff_ref=Eoff_m J  Err_ref=0.5e-3 J  Iref=Ion_sw_loss_m A  Vref=Voff_sw_loss_m V  ki=1  kv=1  Vth_off=50 V  Vth_on=25 V  V_sm=10 V  tau_s=100e-9 s  tau_v=10e-6 s  tau_p=50e-6 s  i_eps=1e-3 A  v_eps=1e-3 V  v_specify=off  v_priority=None  v=0 V  v_nominal_specify=off  v_nominal_value=1  v_nominal_unit=V  i_specify=off  i_priority=None  i=0 A  i_nominal_specify=off  i_nominal_value=1  i_nominal_unit=A  ich_specify=off  ich_priority=None  ich=0 A  ich_nominal_specify=off  ich_nominal_value=1  ich_nominal_unit=A  ichp_specify=off  ichp_priority=None  ichp=0 A  ichp_nominal_specify=off  ichp_nominal_value=1  ichp_nominal_unit=A  idio_specify=off  idio_priority=None  idio=0 A  idio_nominal_specify=off  idio_nominal_value=1  idio_nominal_unit=A  vfd_specify=off  vfd_priority=None  vfd=0 V  vfd_nominal_specify=off  vfd_nominal_value=1  vfd_nominal_unit=V  ith_specify=off  ith_priority=None  ith=0 A  ith_nominal_specify=off  ith_nominal_value=1  ith_nominal_unit=A  idh_specify=off  idh_priority=None  idh=0 A  idh_nominal_specify=off  idh_nominal_value=1  idh_nominal_unit=A  vbl_specify=off  vbl_priority=None  vbl=600 V  vbl_nominal_specify=off  vbl_nominal_value=1  vbl_nominal_unit=V  hb_specify=off  hb_priority=None  hb=0  hb_nominal_specify=off  hb_nominal_value=1  hb_nominal_unit=1  Gch_specify=off  Gch_priority=None  Gch=0 S  Gch_nominal_specify=off  Gch_nominal_value=1  Gch_nominal_unit=S  gl_specify=off  gl_priority=None  gl=0  gl_nominal_specify=off  gl_nominal_value=1  gl_nominal_unit=1  Rds_specify=off  Rds_priority=None  Rds=1e-3 Ohm  Rds_nominal_specify=off  Rds_nominal_value=1  Rds_nominal_unit=Ohm  xr_specify=off  xr_priority=None  xr=1  xr_nominal_specify=off  xr_nominal_value=1  xr_nominal_unit=1  Eot_specify=off  Eot_priority=None  Eot=0 J  Eot_nominal_specify=off  Eot_nominal_value=1  Eot_nominal_unit=J  Eod_specify=off  Eod_priority=None  Eod=0 J  Eod_nominal_specify=off  Eod_nominal_value=1  Eod_nominal_unit=J  Pswt_specify=off  Pswt_priority=None  Pswt=0 W  Pswt_nominal_specify=off  Pswt_nominal_value=1  Pswt_nominal_unit=W  Pswd_specify=off  Pswd_priority=None  Pswd=0 W  Pswd_nominal_specify=off  Pswd_nominal_value=1  Pswd_nominal_unit=W  Pct_specify=off  Pct_priority=None  Pct=0 W  Pct_nominal_specify=off  Pct_nominal_value=1  Pct_nominal_unit=W  Pcd_specify=off  Pcd_priority=None  Pcd=0 W  Pcd_nominal_specify=off  Pcd_nominal_value=1  Pcd_nominal_unit=W  Qt_specify=off  Qt_priority=None  Qt=0 W  Qt_nominal_specify=off  Qt_nominal_value=1  Qt_nominal_unit=W  Qd_specify=off  Qd_priority=None  Qd=0 W  Qd_nominal_specify=off  Qd_nominal_value=1  Qd_nominal_unit=W  Eqt_specify=off  Eqt_priority=None  Eqt=0 J  Eqd_specify=off  Eqd_priority=None  Eqd=0 J
  G : PMIOPort  Side=Left
  H : PMIOPort  Port=2  Side=Left
  D : PMIOPort  Port=3  Side=Left
  S : PMIOPort  Port=4  Side=Right
  connections:
  mos_simple_2th/LConn1 -- D/RConn1
  mos_simple_2th/RConn1 -- S/RConn1
  mos_simple_2th/LConn3 -- G/RConn1
  mos_simple_2th/LConn2 -- mos_simple_2th/RConn2 -- H/RConn1
  PS Terminator/LConn1 -- mos_simple_2th/RConn3
  PS Terminator1/LConn1 -- mos_simple_2th/RConn4
  PS Terminator2/LConn1 -- mos_simple_2th/RConn5
  PS Terminator3/LConn1 -- mos_simple_2th/RConn6

== system sst_cllc_dcx/dcdc_cllc_modA/dc//dc with galvanic isolation/full-bridge 1/full-full_bridge_ssc_mosfet_based/full_bridge_ssc_mosfet_based/mosfet_thermal_2/mos_simple_2th ==
  PS Terminator{,1..3} (4 alike) : fl_lib/Physical Signals/Sinks/PS Terminator
  mos_simple_2th : mos_simple_2th_lib/MOS_SIMPLE_2TH Simplified power MOSFET + antiparallel diode, two thermal ports  Rds_on=Rds_on_m Ohm  alpha_R=0 1/K  Tj_ref=398.15 K  Roff=1e7 Ohm  Vf=Vdon_diode_m V  Rd=Rdon_diode_m Ohm  two_die=1  G_th=0.5  Eon_ref=Eon_m J  Eoff_ref=Eoff_m J  Err_ref=0.5e-3 J  Iref=Ion_sw_loss_m A  Vref=Voff_sw_loss_m V  ki=1  kv=1  Vth_off=50 V  Vth_on=25 V  V_sm=10 V  tau_s=100e-9 s  tau_v=10e-6 s  tau_p=50e-6 s  i_eps=1e-3 A  v_eps=1e-3 V  v_specify=off  v_priority=None  v=0 V  v_nominal_specify=off  v_nominal_value=1  v_nominal_unit=V  i_specify=off  i_priority=None  i=0 A  i_nominal_specify=off  i_nominal_value=1  i_nominal_unit=A  ich_specify=off  ich_priority=None  ich=0 A  ich_nominal_specify=off  ich_nominal_value=1  ich_nominal_unit=A  ichp_specify=off  ichp_priority=None  ichp=0 A  ichp_nominal_specify=off  ichp_nominal_value=1  ichp_nominal_unit=A  idio_specify=off  idio_priority=None  idio=0 A  idio_nominal_specify=off  idio_nominal_value=1  idio_nominal_unit=A  vfd_specify=off  vfd_priority=None  vfd=0 V  vfd_nominal_specify=off  vfd_nominal_value=1  vfd_nominal_unit=V  ith_specify=off  ith_priority=None  ith=0 A  ith_nominal_specify=off  ith_nominal_value=1  ith_nominal_unit=A  idh_specify=off  idh_priority=None  idh=0 A  idh_nominal_specify=off  idh_nominal_value=1  idh_nominal_unit=A  vbl_specify=off  vbl_priority=None  vbl=600 V  vbl_nominal_specify=off  vbl_nominal_value=1  vbl_nominal_unit=V  hb_specify=off  hb_priority=None  hb=0  hb_nominal_specify=off  hb_nominal_value=1  hb_nominal_unit=1  Gch_specify=off  Gch_priority=None  Gch=0 S  Gch_nominal_specify=off  Gch_nominal_value=1  Gch_nominal_unit=S  gl_specify=off  gl_priority=None  gl=0  gl_nominal_specify=off  gl_nominal_value=1  gl_nominal_unit=1  Rds_specify=off  Rds_priority=None  Rds=1e-3 Ohm  Rds_nominal_specify=off  Rds_nominal_value=1  Rds_nominal_unit=Ohm  xr_specify=off  xr_priority=None  xr=1  xr_nominal_specify=off  xr_nominal_value=1  xr_nominal_unit=1  Eot_specify=off  Eot_priority=None  Eot=0 J  Eot_nominal_specify=off  Eot_nominal_value=1  Eot_nominal_unit=J  Eod_specify=off  Eod_priority=None  Eod=0 J  Eod_nominal_specify=off  Eod_nominal_value=1  Eod_nominal_unit=J  Pswt_specify=off  Pswt_priority=None  Pswt=0 W  Pswt_nominal_specify=off  Pswt_nominal_value=1  Pswt_nominal_unit=W  Pswd_specify=off  Pswd_priority=None  Pswd=0 W  Pswd_nominal_specify=off  Pswd_nominal_value=1  Pswd_nominal_unit=W  Pct_specify=off  Pct_priority=None  Pct=0 W  Pct_nominal_specify=off  Pct_nominal_value=1  Pct_nominal_unit=W  Pcd_specify=off  Pcd_priority=None  Pcd=0 W  Pcd_nominal_specify=off  Pcd_nominal_value=1  Pcd_nominal_unit=W  Qt_specify=off  Qt_priority=None  Qt=0 W  Qt_nominal_specify=off  Qt_nominal_value=1  Qt_nominal_unit=W  Qd_specify=off  Qd_priority=None  Qd=0 W  Qd_nominal_specify=off  Qd_nominal_value=1  Qd_nominal_unit=W  Eqt_specify=off  Eqt_priority=None  Eqt=0 J  Eqd_specify=off  Eqd_priority=None  Eqd=0 J
  G : PMIOPort  Side=Left
  H : PMIOPort  Port=2  Side=Left
  D : PMIOPort  Port=3  Side=Left
  S : PMIOPort  Port=4  Side=Right
  connections:
  mos_simple_2th/LConn1 -- D/RConn1
  mos_simple_2th/RConn1 -- S/RConn1
  mos_simple_2th/LConn3 -- G/RConn1
  mos_simple_2th/LConn2 -- mos_simple_2th/RConn2 -- H/RConn1
  PS Terminator/LConn1 -- mos_simple_2th/RConn3
  PS Terminator1/LConn1 -- mos_simple_2th/RConn4
  PS Terminator2/LConn1 -- mos_simple_2th/RConn5
  PS Terminator3/LConn1 -- mos_simple_2th/RConn6

== system sst_cllc_dcx/dcdc_cllc_modA/dc//dc with galvanic isolation/full-bridge 1/full-full_bridge_ssc_mosfet_based/full_bridge_ssc_mosfet_based/mosfet_thermal_3/mos_simple_2th ==
  PS Terminator{,1..3} (4 alike) : fl_lib/Physical Signals/Sinks/PS Terminator
  mos_simple_2th : mos_simple_2th_lib/MOS_SIMPLE_2TH Simplified power MOSFET + antiparallel diode, two thermal ports  Rds_on=Rds_on_m Ohm  alpha_R=0 1/K  Tj_ref=398.15 K  Roff=1e7 Ohm  Vf=Vdon_diode_m V  Rd=Rdon_diode_m Ohm  two_die=1  G_th=0.5  Eon_ref=Eon_m J  Eoff_ref=Eoff_m J  Err_ref=0.5e-3 J  Iref=Ion_sw_loss_m A  Vref=Voff_sw_loss_m V  ki=1  kv=1  Vth_off=50 V  Vth_on=25 V  V_sm=10 V  tau_s=100e-9 s  tau_v=10e-6 s  tau_p=50e-6 s  i_eps=1e-3 A  v_eps=1e-3 V  v_specify=off  v_priority=None  v=0 V  v_nominal_specify=off  v_nominal_value=1  v_nominal_unit=V  i_specify=off  i_priority=None  i=0 A  i_nominal_specify=off  i_nominal_value=1  i_nominal_unit=A  ich_specify=off  ich_priority=None  ich=0 A  ich_nominal_specify=off  ich_nominal_value=1  ich_nominal_unit=A  ichp_specify=off  ichp_priority=None  ichp=0 A  ichp_nominal_specify=off  ichp_nominal_value=1  ichp_nominal_unit=A  idio_specify=off  idio_priority=None  idio=0 A  idio_nominal_specify=off  idio_nominal_value=1  idio_nominal_unit=A  vfd_specify=off  vfd_priority=None  vfd=0 V  vfd_nominal_specify=off  vfd_nominal_value=1  vfd_nominal_unit=V  ith_specify=off  ith_priority=None  ith=0 A  ith_nominal_specify=off  ith_nominal_value=1  ith_nominal_unit=A  idh_specify=off  idh_priority=None  idh=0 A  idh_nominal_specify=off  idh_nominal_value=1  idh_nominal_unit=A  vbl_specify=off  vbl_priority=None  vbl=600 V  vbl_nominal_specify=off  vbl_nominal_value=1  vbl_nominal_unit=V  hb_specify=off  hb_priority=None  hb=0  hb_nominal_specify=off  hb_nominal_value=1  hb_nominal_unit=1  Gch_specify=off  Gch_priority=None  Gch=0 S  Gch_nominal_specify=off  Gch_nominal_value=1  Gch_nominal_unit=S  gl_specify=off  gl_priority=None  gl=0  gl_nominal_specify=off  gl_nominal_value=1  gl_nominal_unit=1  Rds_specify=off  Rds_priority=None  Rds=1e-3 Ohm  Rds_nominal_specify=off  Rds_nominal_value=1  Rds_nominal_unit=Ohm  xr_specify=off  xr_priority=None  xr=1  xr_nominal_specify=off  xr_nominal_value=1  xr_nominal_unit=1  Eot_specify=off  Eot_priority=None  Eot=0 J  Eot_nominal_specify=off  Eot_nominal_value=1  Eot_nominal_unit=J  Eod_specify=off  Eod_priority=None  Eod=0 J  Eod_nominal_specify=off  Eod_nominal_value=1  Eod_nominal_unit=J  Pswt_specify=off  Pswt_priority=None  Pswt=0 W  Pswt_nominal_specify=off  Pswt_nominal_value=1  Pswt_nominal_unit=W  Pswd_specify=off  Pswd_priority=None  Pswd=0 W  Pswd_nominal_specify=off  Pswd_nominal_value=1  Pswd_nominal_unit=W  Pct_specify=off  Pct_priority=None  Pct=0 W  Pct_nominal_specify=off  Pct_nominal_value=1  Pct_nominal_unit=W  Pcd_specify=off  Pcd_priority=None  Pcd=0 W  Pcd_nominal_specify=off  Pcd_nominal_value=1  Pcd_nominal_unit=W  Qt_specify=off  Qt_priority=None  Qt=0 W  Qt_nominal_specify=off  Qt_nominal_value=1  Qt_nominal_unit=W  Qd_specify=off  Qd_priority=None  Qd=0 W  Qd_nominal_specify=off  Qd_nominal_value=1  Qd_nominal_unit=W  Eqt_specify=off  Eqt_priority=None  Eqt=0 J  Eqd_specify=off  Eqd_priority=None  Eqd=0 J
  G : PMIOPort  Side=Left
  H : PMIOPort  Port=2  Side=Left
  D : PMIOPort  Port=3  Side=Left
  S : PMIOPort  Port=4  Side=Right
  connections:
  mos_simple_2th/LConn1 -- D/RConn1
  mos_simple_2th/RConn1 -- S/RConn1
  mos_simple_2th/LConn3 -- G/RConn1
  mos_simple_2th/LConn2 -- mos_simple_2th/RConn2 -- H/RConn1
  PS Terminator/LConn1 -- mos_simple_2th/RConn3
  PS Terminator1/LConn1 -- mos_simple_2th/RConn4
  PS Terminator2/LConn1 -- mos_simple_2th/RConn5
  PS Terminator3/LConn1 -- mos_simple_2th/RConn6
